simulink model "sm_car"  (R2025a)
settings: Solver=ode23t  StartTime=0.0  StopTime=400  MaxStep=0.4  RelTol=1e-3  AbsTol=1e-3  EnableMultiTasking=on
PreLoadFcn:
  | % Due to usability issue in Repeating Sequence block
  | warning('off','Simulink:Masking:Invalid');
  | 
  | % Eliminate unnecessary warnings in inactive variants
  | % Warnings generated only if you click through inactive variant
  | warning('off','MATLAB:nonExistentField');
  | warning('off','Simulink:Parameters:BlkParamUndefined');
PostLoadFcn:
  | set_param([bdroot '/Vehicle'],'popup_trailer','Off')
  | warning('off','sm:sli:setup:compile:LocalSolverNotSupported')
  | %sm_car_config_maneuver(bdroot,'WOT Braking');
  | sm_car_config_vehicle(bdroot,'false');
  | sm_car_config_logging(bdroot);
InitFcn:
  | sm_car_config_camera;
  | Vehicle = sm_car_vehcfg_checkConfig(Vehicle);
  | sm_car_check_tire_model(bdroot);
StartFcn:
  | tic;
StopFcn:
  | Elapsed_Sim_Time = toc;
  | % disp(['Elapsed Sim Time = ' num2str(Elapsed_Sim_Time)]);
undefined symbols (not defined in the file): Axle1D, AxleIn, Camera, Control, Driver, Free, Init, Maneuver, Pedal, RaceFix, RaceSpin, Scene, ShaftL1, ShaftL2, ShaftR1, ShaftR2, Soft, Stiff, Visual, X, xy_data_car_side, Y, Z
libraries: sm_lib x1546, nesl_utility x528, fl_lib x480, SimscapeFluids_lib x61, sdl_lib x49, simulink x29, ee_lib x7, simulink_extras x6, Linkage_Systems x4, Tire_1x2x x4, AntiRollBar_Systems x2, Linkage_Decoupled x2
(part 46 of 79)

== system sm_car/Vehicle/Vehicle/Chassis/Spring/Decoupled/Spring A2 Heave/AirOilPiston/Sensor Motion Strut ==
  Motion Sensor : fl_lib/Mechanical/Mechanical Sensors/Ideal Translational Motion Sensor  reference=foundation.enum.MeasurementReference.difference  acceleration_port=false  velocity_port=true  position_port=true  offset=spr_len0 m
  PS-Simulink Converter : nesl_utility/PS-Simulink Converter  PhysicalDomain=network_engine_domain  SubClassName=ps_output  LeftPortType=input  RightPortType=output  PseudoPeriodic=off  Frequencies=[]  VectorFormat=inherit  Unit=inherit  AffineConversion=off
  PS-Simulink Converter1 : nesl_utility/PS-Simulink Converter  PhysicalDomain=network_engine_domain  SubClassName=ps_output  LeftPortType=input  RightPortType=output  PseudoPeriodic=off  Frequencies=[]  VectorFormat=inherit  Unit=m  AffineConversion=off
  C : PMIOPort  Side=Left
  R : PMIOPort  Port=2  Side=Left
  P : Outport
  V : Outport  Port=2
  wires:
  PS-Simulink Converter1/1 -> P/1
  PS-Simulink Converter/1 -> V/1
  connections:
  Motion Sensor/RConn3 -- PS-Simulink Converter1/LConn1
  PS-Simulink Converter/LConn1 -- Motion Sensor/RConn2
  Motion Sensor/RConn1 -- C/RConn1
  Motion Sensor/LConn1 -- R/RConn1

== system sm_car/Vehicle/Vehicle/Chassis/Spring/Decoupled/Spring A2 Heave/AirOilPiston/Sensor Spring Force ==
  Force Spring : fl_lib/Mechanical/Mechanical Sensors/Ideal Force Sensor
  PS-Simulink Converter1 : nesl_utility/PS-Simulink Converter  PhysicalDomain=network_engine_domain  SubClassName=ps_output  LeftPortType=input  RightPortType=output  PseudoPeriodic=off  Frequencies=[]  VectorFormat=1-D array  Unit=N  AffineConversion=off
  R : PMIOPort  Side=Left
  C : PMIOPort  Port=2  Side=Right
  f : Outport
  wires:
  PS-Simulink Converter1/1 -> f/1
  connections:
  Force Spring/RConn1 -- C/RConn1
  PS-Simulink Converter1/LConn1 -- Force Spring/RConn2
  Force Spring/LConn1 -- R/RConn1

== system sm_car/Vehicle/Vehicle/Chassis/Spring/Decoupled/Spring A2 Heave/AirOilPiston/Sensor Strut Pressure ==
  PS-Simulink Converter7 : nesl_utility/PS-Simulink Converter  PhysicalDomain=network_engine_domain  SubClassName=ps_output  LeftPortType=input  RightPortType=output  PseudoPeriodic=off  Frequencies=[]  VectorFormat=inherit  Unit=MPa  AffineConversion=off
  Sensor Pressure : fl_lib/Isothermal Liquid/Sensors/Pressure Sensor (IL)  pressure_measure=foundation.enum.pressure_measure.gauge
      settings: InternalSimscapePortConfiguration="{\"Bottom\":[],\"Left\":[{\"id\":\"A\",\"label\":\"A\",\"type\":\"foundation.isothermal_liquid.isothermal_liquid\"}],\"Right\":[{\"id\":\"Pg\",\"label\":\"Pg\",\"type\":\"output\"}],\"Top\":[]}"
  A : PMIOPort  Side=Left
  P : Outport
  wires:
  PS-Simulink Converter7/1 -> P/1
  connections:
  Sensor Pressure/RConn1 -- PS-Simulink Converter7/LConn1
  Sensor Pressure/LConn1 -- A/RConn1

== system sm_car/Vehicle/Vehicle/Chassis/Spring/Decoupled/Spring A2 Roll/AirOilPiston/Damper ==
  note: Constant Volume Chambers added for robust simulation and flexible initialization.
  ctrl : Inport
  CVC Comp : fl_lib/Isothermal Liquid/Elements/Constant Volume Chamber (IL)  volume=0.0001 m^3  p_I_specify=on  p_I_priority=Low  p_I=0.101325 MPa  p_I_nominal_specify=off  p_I_nominal_value=1  p_I_nominal_unit=MPa
      settings: InternalSimscapePortConfiguration="{\"Bottom\":[],\"Left\":[{\"id\":\"A\",\"label\":\"A\",\"type\":\"foundation.isothermal_liquid.isothermal_liquid\"}],\"Right\":[],\"Top\":[]}"
  CVC Reb : fl_lib/Isothermal Liquid/Elements/Constant Volume Chamber (IL)  volume=0.0001 m^3  p_I_specify=on  p_I_priority=Low  p_I=0.101325 MPa  p_I_nominal_specify=off  p_I_nominal_value=1  p_I_nominal_unit=MPa
      settings: InternalSimscapePortConfiguration="{\"Bottom\":[],\"Left\":[{\"id\":\"A\",\"label\":\"A\",\"type\":\"foundation.isothermal_liquid.isothermal_liquid\"}],\"Right\":[],\"Top\":[]}"
  CVC Spring : fl_lib/Isothermal Liquid/Elements/Constant Volume Chamber (IL)  volume=0.0001 m^3  p_I_specify=on  p_I_priority=Low  p_I=0.101325 MPa  p_I_nominal_specify=off  p_I_nominal_value=1  p_I_nominal_unit=MPa
      settings: InternalSimscapePortConfiguration="{\"Bottom\":[],\"Left\":[{\"id\":\"A\",\"label\":\"A\",\"type\":\"foundation.isothermal_liquid.isothermal_liquid\"}],\"Right\":[],\"Top\":[]}"
  CVC Strut : fl_lib/Isothermal Liquid/Elements/Constant Volume Chamber (IL)  volume=0.0001 m^3  p_I_specify=on  p_I_priority=Low  p_I=0.101325 MPa  p_I_nominal_specify=off  p_I_nominal_value=1  p_I_nominal_unit=MPa
      settings: InternalSimscapePortConfiguration="{\"Bottom\":[],\"Left\":[{\"id\":\"A\",\"label\":\"A\",\"type\":\"foundation.isothermal_liquid.isothermal_liquid\"}],\"Right\":[],\"Top\":[]}"
  CVD Actuator : SimscapeFluids_lib/Valve Actuators/Proportional Valve Actuator  gain=1 m  time_constant=dpr_cvdvalve_act_ts s  valve_stroke=1 m
      settings: InternalSimscapePortConfiguration="{\"Bottom\":[],\"Left\":[{\"id\":\"A\",\"label\":\"A\",\"type\":\"input\"}],\"Right\":[{\"id\":\"S\",\"label\":\"S\",\"type\":\"output\"}],\"Top\":[]}"
  CVD Valve : SimscapeFluids_lib/Isothermal Liquid/Valves & Orifices/Flow Control Valves/Pressure-Compensated Flow Control Valve (IL)  orifice_spec=fluids.isothermal_liquid.valves_orifices.orifices.enum.orifice_spec.table1D_area_opening  S_min=0 m  del_S=1 m  area_max=A_damp_blow_comp m^2  S_TLU=dpr_cvdvalve_cmpos m  orifice_area_TLU=dpr_cvdvalve_orifice_area m^2  S_vol_flow_TLU=[0, .002, .004, .007, .017] m  p_diff_TLU=[.3, .5, .7] MPa  vol_flow_TLU=1e-3 * [1.7e-05, 2e-05, 2.6e-05; .0035, .0045, .0053; .7, .9, 1.06; 1.96, 2.5, 3; 6, 7.7, 9.13] m^3/s  p_diff_orifice=dpr_cvdvalve_orifice_pdiff bar  p_range=dpr_cvdvalve_pcv_prange bar  area_max_compensator=dpr_cvdvalve_pcv_areamax m^2  area_leak=dpr_cvdvalve_arealeak m^2  Cd=dpr_cvdvalve_cd  Re_c=150  smoothing_factor=0.01
      settings: InternalSimscapePortConfiguration="{\"Bottom\":[],\"Left\":[{\"id\":\"S\",\"label\":\"S\",\"type\":\"input\"},{\"id\":\"A\",\"label\":\"A\",\"type\":\"foundation.isothermal_liquid.isothermal_liquid\"}],\"Right\":[{\"id\":\"B\",\"label\":\"B\",\"type\":\"foundation.isothermal_liquid.isothermal_liquid\"}],\"Top\":[]}"
  Orifice Low Speed : SimscapeFluids_lib/Isothermal Liquid/Valves & Orifices/Orifices/Orifice (IL)  orifice_type=foundation.enum.constant_variable.constant  constant_orifice_spec=fluids.isothermal_liquid.valves_orifices.orifices.enum.constant_orifice_spec.table1D_volflow_pressure  variable_orifice_spec=fluids.isothermal_liquid.valves_orifices.orifices.enum.orifice_spec.linear  orifice_area_constant=1e-3 m^2  p_diff_TLU_constant=p_diff_TLU_constant MPa  vol_flow_TLU_constant=vol_flow_TLU_constant m^3/s  S_min=0 m  del_S=5e-3 m  open_orientation=fluids.isothermal_liquid.valves_orifices.orifices.enum.orifice_orientation.positive  area_max=1e-4 m^2  area_leak=1e-10 m^2  S_TLU=[0, .002, .004, .007, .017] m  orifice_area_TLU=[1e-09, 2.0352e-07, 4.0736e-05, .00011438, .00034356] m^2  area=inf m^2  Cd=0.64  Re_c=150  smoothing_factor=0.01  pressure_recovery=false  S_vol_flow_TLU=[0, .002, .004, .007, .017] m  p_diff_TLU=[.3, .5, .7] MPa  vol_flow_TLU=1e-3 * [1.7e-05, 2e-05, 2.6e-05; .0035, .0045, .0053; .7, .9, 1.06; 1.96, 2.5, 3; 6, 7.7, 9.13] m^3/s
      settings: InternalSimscapePortConfiguration="{\"Bottom\":[],\"Left\":[{\"id\":\"A\",\"label\":\"A\",\"type\":\"foundation.isothermal_liquid.isothermal_liquid\"}],\"Right\":[{\"id\":\"B\",\"label\":\"B\",\"type\":\"foundation.isothermal_liquid.isothermal_liquid\"}],\"Top\":[]}"
  PRV Comp : SimscapeFluids_lib/Isothermal Liquid/Valves & Orifices/Pressure Control Valves/Pressure Relief Valve (IL)  set_pressure_spec=foundation.enum.constant_controlled.constant  opening_spec=fluids.isothermal_liquid.valves_orifices.enum.PressureOpeningSpec.Linear  pressure_spec=fluids.isothermal_liquid.valves_orifices.enum.pressure_control_spec.dp  p_set_gauge=0.1 MPa  p_set_differential=dpr_prv_psetdiff_comp MPa  p_range=dpr_prv_prange_reb MPa  area_max=dpr_prv_areamax_comp m^2  area_leak=1e-10 m^2  p_diff_TLU=[0.2 : 0.2 : 1.2] MPa  p_gauge_TLU=[0.2 : 0.2 : 1.2] MPa  valve_area_TLU=[1e-10, 2e-06, 4e-06, 6e-06, 8e-06, 1e-05] m^2  vol_flow_TLU=[1e-09, 3.6e-05, 8.9e-05, .00015, .00023, .00031] m^3/s  area=inf m^2  Cd=dpr_prv_cd_comp  Re_c=150  smoothing_factor=0.05  pressure_recovery=simscape.enum.onoff.off  opening_dynamics=false  tau=0.005 s
      settings: InternalSimscapePortConfiguration="{\"Bottom\":[],\"Left\":[{\"id\":\"A\",\"label\":\"A\",\"type\":\"foundation.isothermal_liquid.isothermal_liquid\"}],\"Right\":[{\"id\":\"B\",\"label\":\"B\",\"type\":\"foundation.isothermal_liquid.isothermal_liquid\"}],\"Top\":[]}"
  PRV Reb : SimscapeFluids_lib/Isothermal Liquid/Valves & Orifices/Pressure Control Valves/Pressure Relief Valve (IL)  set_pressure_spec=foundation.enum.constant_controlled.constant  opening_spec=fluids.isothermal_liquid.valves_orifices.enum.PressureOpeningSpec.Linear  pressure_spec=fluids.isothermal_liquid.valves_orifices.enum.pressure_control_spec.dp  p_set_gauge=0.1 MPa  p_set_differential=dpr_prv_psetdiff_reb MPa  p_range=dpr_prv_prange_comp MPa  area_max=dpr_prv_areamax_reb m^2  area_leak=1e-10 m^2  p_diff_TLU=[0.2 : 0.2 : 1.2] MPa  p_gauge_TLU=[0.2 : 0.2 : 1.2] MPa  valve_area_TLU=[1e-10, 2e-06, 4e-06, 6e-06, 8e-06, 1e-05] m^2  vol_flow_TLU=[1e-09, 3.6e-05, 8.9e-05, .00015, .00023, .00031] m^3/s  area=inf m^2  Cd=dpr_prv_cd_reb  Re_c=150  smoothing_factor=0.05  pressure_recovery=simscape.enum.onoff.off  opening_dynamics=false  tau=0.005 s
      settings: InternalSimscapePortConfiguration="{\"Bottom\":[],\"Left\":[{\"id\":\"A\",\"label\":\"A\",\"type\":\"foundation.isothermal_liquid.isothermal_liquid\"}],\"Right\":[{\"id\":\"B\",\"label\":\"B\",\"type\":\"foundation.isothermal_liquid.isothermal_liquid\"}],\"Top\":[]}"
  PS-Simulink Converter{,1,4..5} (4 alike) : nesl_utility/PS-Simulink Converter  PhysicalDomain=network_engine_domain  SubClassName=ps_output  LeftPortType=input  RightPortType=output  PseudoPeriodic=off  Frequencies=[]  VectorFormat=inherit  Unit=inherit  AffineConversion=off
  PS-Simulink Converter2 : nesl_utility/PS-Simulink Converter  PhysicalDomain=network_engine_domain  SubClassName=ps_output  LeftPortType=input  RightPortType=output  PseudoPeriodic=off  Frequencies=[]  VectorFormat=inherit  Unit=MPa  AffineConversion=off
  PS-Simulink Converter3 : nesl_utility/PS-Simulink Converter  PhysicalDomain=network_engine_domain  SubClassName=ps_output  LeftPortType=input  RightPortType=output  PseudoPeriodic=off  Frequencies=[]  VectorFormat=inherit  Unit=MPa  AffineConversion=off
  Restr Comp : fl_lib/Isothermal Liquid/Elements/Local Restriction (IL)  restriction_type=foundation.enum.restriction_type.fixed  restriction_area=dpr_restrarea_comp m^2  min_area=1.3273e-06 m^2  max_area=0.005 m^2  area=inf m^2  Cd=dpr_cd_comp  Re_c=150  pressure_recovery=true
      settings: InternalSimscapePortConfiguration="{\"Bottom\":[],\"Left\":[{\"id\":\"A\",\"label\":\"A\",\"type\":\"foundation.isothermal_liquid.isothermal_liquid\"}],\"Right\":[{\"id\":\"B\",\"label\":\"B\",\"type\":\"foundation.isothermal_liquid.isothermal_liquid\"}],\"Top\":[]}"
  Restr Reb : fl_lib/Isothermal Liquid/Elements/Local Restriction (IL)  restriction_type=foundation.enum.restriction_type.fixed  restriction_area=dpr_restrarea_reb m^2  min_area=1.3273e-06 m^2  max_area=0.005 m^2  area=inf m^2  Cd=dpr_cd_reb  Re_c=150  pressure_recovery=true
      settings: InternalSimscapePortConfiguration="{\"Bottom\":[],\"Left\":[{\"id\":\"A\",\"label\":\"A\",\"type\":\"foundation.isothermal_liquid.isothermal_liquid\"}],\"Right\":[{\"id\":\"B\",\"label\":\"B\",\"type\":\"foundation.isothermal_liquid.isothermal_liquid\"}],\"Top\":[]}"
  Sensor CVD Flow : fl_lib/Isothermal Liquid/Sensors/Flow Rate Sensor (IL)  sensor_type=foundation.enum.mass_volumetric_sensor.mass
      settings: InternalSimscapePortConfiguration="{\"Bottom\":[],\"Left\":[{\"id\":\"A\",\"label\":\"A\",\"type\":\"foundation.isothermal_liquid.isothermal_liquid\"}],\"Right\":[{\"id\":\"B\",\"label\":\"B\",\"type\":\"foundation.isothermal_liquid.isothermal_liquid\"},{\"id\":\"M\",\"label\":\"M\",\"type\":\"output\"}],\"Top\":[]}"
  Sensor Flow Orifice : fl_lib/Isothermal Liquid/Sensors/Flow Rate Sensor (IL)  sensor_type=foundation.enum.mass_volumetric_sensor.mass
      settings: InternalSimscapePortConfiguration="{\"Bottom\":[],\"Left\":[{\"id\":\"A\",\"label\":\"A\",\"type\":\"foundation.isothermal_liquid.isothermal_liquid\"}],\"Right\":[{\"id\":\"B\",\"label\":\"B\",\"type\":\"foundation.isothermal_liquid.isothermal_liquid\"},{\"id\":\"M\",\"label\":\"M\",\"type\":\"output\"}],\"Top\":[]}"
  Sensor Flow Comp : fl_lib/Isothermal Liquid/Sensors/Flow Rate Sensor (IL)  sensor_type=foundation.enum.mass_volumetric_sensor.mass
      settings: InternalSimscapePortConfiguration="{\"Bottom\":[],\"Left\":[{\"id\":\"A\",\"label\":\"A\",\"type\":\"foundation.isothermal_liquid.isothermal_liquid\"}],\"Right\":[{\"id\":\"B\",\"label\":\"B\",\"type\":\"foundation.isothermal_liquid.isothermal_liquid\"},{\"id\":\"M\",\"label\":\"M\",\"type\":\"output\"}],\"Top\":[]}"
  Sensor Flow Reb : fl_lib/Isothermal Liquid/Sensors/Flow Rate Sensor (IL)  sensor_type=foundation.enum.mass_volumetric_sensor.mass
      settings: InternalSimscapePortConfiguration="{\"Bottom\":[],\"Left\":[{\"id\":\"A\",\"label\":\"A\",\"type\":\"foundation.isothermal_liquid.isothermal_liquid\"}],\"Right\":[{\"id\":\"B\",\"label\":\"B\",\"type\":\"foundation.isothermal_liquid.isothermal_liquid\"},{\"id\":\"M\",\"label\":\"M\",\"type\":\"output\"}],\"Top\":[]}"
  Sensor Pressure Block : fl_lib/Isothermal Liquid/Sensors/Pressure Sensor (IL)  pressure_measure=foundation.enum.pressure_measure.gauge
      settings: InternalSimscapePortConfiguration="{\"Bottom\":[],\"Left\":[{\"id\":\"A\",\"label\":\"A\",\"type\":\"foundation.isothermal_liquid.isothermal_liquid\"}],\"Right\":[{\"id\":\"Pg\",\"label\":\"Pg\",\"type\":\"output\"}],\"Top\":[]}"
  Sensor Pressure Diff : fl_lib/Isothermal Liquid/Sensors/Pressure Sensor (IL)  pressure_measure=foundation.enum.pressure_measure.difference
      settings: InternalSimscapePortConfiguration="{\"Bottom\":[],\"Left\":[{\"id\":\"A\",\"label\":\"A\",\"type\":\"foundation.isothermal_liquid.isothermal_liquid\"}],\"Right\":[{\"id\":\"B\",\"label\":\"B\",\"type\":\"foundation.isothermal_liquid.isothermal_liquid\"},{\"id\":\"P\",\"label\":\"P\",\"type\":\"output\"}],\"Top\":[]}"
  Simulink-PS Converter2 : nesl_utility/Simulink-PS Converter  PhysicalDomain=network_engine_domain  SubClassName=ps_input  LeftPortType=input  RightPortType=output  PseudoPeriodic=off  Frequencies=[]  NoiseDistribution=none  NoiseParameters=[]  Unit=1  AffineConversion=off  FilteringAndDerivatives=provide  SimscapeFilterOrder=1  InputFilterTimeConstant=0.001  UdotUserProvided=0
  Strut : PMIOPort  Side=Left
  Spr : PMIOPort  Port=2  Side=Left
  Bus Element Out : Outport  PortName=m  Element=Pdiff
  Bus Element Out1 : Outport  PortName=m  Element=PBlock
  Bus Element Out2 : Outport  PortName=m  Element=qmReb
  Bus Element Out3 : Outport  PortName=m  Element=qmComp
  Bus Element Out4 : Outport  PortName=m  Element=qmCVD
  Bus Element Out5 : Outport  PortName=m  Element=qmOrifice
  wires:
  ctrl/1 -> Simulink-PS Converter2/1
  PS-Simulink Converter4/1 -> Bus Element Out4/1
  PS-Simulink Converter3/1 -> Bus Element Out1/1
  PS-Simulink Converter2/1 -> Bus Element Out/1
  PS-Simulink Converter1/1 -> Bus Element Out3/1
  PS-Simulink Converter/1 -> Bus Element Out2/1
  PS-Simulink Converter5/1 -> Bus Element Out5/1
  connections:
  Restr Comp/RConn1 -- CVC Comp/LConn1 -- PRV Comp/LConn1
  Restr Reb/RConn1 -- PRV Reb/RConn1 -- CVC Reb/LConn1
  Sensor CVD Flow/RConn2 -- PS-Simulink Converter4/LConn1
  Sensor CVD Flow/LConn1 -- CVD Valve/RConn1
  CVD Valve/LConn1 -- CVD Actuator/RConn1
  Sensor Pressure Diff/LConn1 -- Restr Reb/LConn1 -- Restr Comp/LConn1 -- Orifice Low Speed/LConn1 -- CVC Strut/LConn1 -- CVD Valve/LConn2 -- Strut/RConn1
  Sensor Pressure Block/RConn1 -- PS-Simulink Converter3/LConn1
  Sensor Pressure Diff/RConn2 -- PS-Simulink Converter2/LConn1
  CVD Actuator/LConn1 -- Simulink-PS Converter2/RConn1
  Sensor Flow Comp/RConn2 -- PS-Simulink Converter1/LConn1
  PRV Comp/RConn1 -- Sensor Flow Comp/LConn1
  PS-Simulink Converter/LConn1 -- Sensor Flow Reb/RConn2
  Sensor Flow Reb/LConn1 -- PRV Reb/LConn1
  Sensor CVD Flow/RConn1 -- Sensor Flow Orifice/RConn1 -- Sensor Flow Reb/RConn1 -- Sensor Flow Comp/RConn1 -- Sensor Pressure Diff/RConn1 -- Sensor Pressure Block/LConn1 -- CVC Spring/LConn1 -- Spr/RConn1
  Orifice Low Speed/RConn1 -- Sensor Flow Orifice/LConn1
  PS-Simulink Converter5/LConn1 -- Sensor Flow Orifice/RConn2

== system sm_car/Vehicle/Vehicle/Chassis/Spring/Decoupled/Spring A2 Roll/AirOilPiston/NC ==
  c : Inport
  Data Type Conversion : DataTypeConversion  SaturateOnIntegerOverflow=off  RndMeth=Floor
  NOT : Logic  Operator=NOT  IconShape=distinctive  AllPortsSameDT=off  OutDataTypeStr=boolean
  Simulink-PS Converter2 : nesl_utility/Simulink-PS Converter  PhysicalDomain=network_engine_domain  SubClassName=ps_input  LeftPortType=input  RightPortType=output  PseudoPeriodic=off  Frequencies=[]  NoiseDistribution=none  NoiseParameters=[]  Unit=1  AffineConversion=off  FilteringAndDerivatives=provide  SimscapeFilterOrder=1  InputFilterTimeConstant=0.001  UdotUserProvided=0
  S : PMIOPort  Side=Right
  wires:
  Data Type Conversion/1 -> Simulink-PS Converter2/1  "GasSprStiff"
  c/1 -> NOT/1
  NOT/1 -> Data Type Conversion/1
  connections:
  Simulink-PS Converter2/RConn1 -- S/RConn1

== system sm_car/Vehicle/Vehicle/Chassis/Spring/Decoupled/Spring A2 Roll/AirOilPiston/Ride Height ==
  ctrlIn : Inport
  ctrlOut : Inport  Port=2
  FCV Actuator Inlet : SimscapeFluids_lib/Valve Actuators/Proportional Valve Actuator  gain=1 m  time_constant=rh_fcv_tfilt_inlet s  valve_stroke=1 m
      settings: InternalSimscapePortConfiguration="{\"Bottom\":[],\"Left\":[{\"id\":\"A\",\"label\":\"A\",\"type\":\"input\"}],\"Right\":[{\"id\":\"S\",\"label\":\"S\",\"type\":\"output\"}],\"Top\":[]}"
  FCV Actuator Outlet : SimscapeFluids_lib/Valve Actuators/Proportional Valve Actuator  gain=1 m  time_constant=rh_fcv_tfilt_outlet s  valve_stroke=1 m
      settings: InternalSimscapePortConfiguration="{\"Bottom\":[],\"Left\":[{\"id\":\"A\",\"label\":\"A\",\"type\":\"input\"}],\"Right\":[{\"id\":\"S\",\"label\":\"S\",\"type\":\"output\"}],\"Top\":[]}"
  FCV Inlet : SimscapeFluids_lib/Isothermal Liquid/Valves & Orifices/Flow Control Valves/Pressure-Compensated Flow Control Valve (IL)  orifice_spec=fluids.isothermal_liquid.valves_orifices.orifices.enum.orifice_spec.table1D_area_opening  S_min=0 m  del_S=1 m  area_max=A_damp_blow_comp m^2  S_TLU=rh_fcv_cmpos_inlet m  orifice_area_TLU=rh_fcv_orificearea_inlet m^2  S_vol_flow_TLU=[0, .002, .004, .007, .017] m  p_diff_TLU=[.3, .5, .7] MPa  vol_flow_TLU=1e-3 * [1.7e-05, 2e-05, 2.6e-05; .0035, .0045, .0053; .7, .9, 1.06; 1.96, 2.5, 3; 6, 7.7, 9.13] m^3/s  p_diff_orifice=rh_fcv_orificepdiff_inlet bar  p_range=rh_fcv_pcprange_inlet bar  area_max_compensator=rh_fcv_pcamax_inlet m^2  area_leak=rh_fcv_arealeak_inlet m^2  Cd=rh_fcv_cd_inlet  Re_c=150  smoothing_factor=rh_fcv_smooth_inlet
      settings: InternalSimscapePortConfiguration="{\"Bottom\":[],\"Left\":[{\"id\":\"S\",\"label\":\"S\",\"type\":\"input\"},{\"id\":\"A\",\"label\":\"A\",\"type\":\"foundation.isothermal_liquid.isothermal_liquid\"}],\"Right\":[{\"id\":\"B\",\"label\":\"B\",\"type\":\"foundation.isothermal_liquid.isothermal_liquid\"}],\"Top\":[]}"
  FCV Outlet : SimscapeFluids_lib/Isothermal Liquid/Valves & Orifices/Flow Control Valves/Pressure-Compensated Flow Control Valve (IL)  orifice_spec=fluids.isothermal_liquid.valves_orifices.orifices.enum.orifice_spec.table1D_area_opening  S_min=0 m  del_S=1 m  area_max=A_damp_blow_comp m^2  S_TLU=rh_fcv_cmpos_outlet m  orifice_area_TLU=rh_fcv_orificearea_outlet m^2  S_vol_flow_TLU=[0, .002, .004, .007, .017] m  p_diff_TLU=[.3, .5, .7] MPa  vol_flow_TLU=1e-3 * [1.7e-05, 2e-05, 2.6e-05; .0035, .0045, .0053; .7, .9, 1.06; 1.96, 2.5, 3; 6, 7.7, 9.13] m^3/s  p_diff_orifice=rh_fcv_orificepdiff_outlet bar  p_range=rh_fcv_pcprange_outlet bar  area_max_compensator=rh_fcv_pcamax_outlet m^2  area_leak=rh_fcv_arealeak_outlet m^2  Cd=rh_fcv_cd_outlet  Re_c=150  smoothing_factor=rh_fcv_smooth_outlet
      settings: InternalSimscapePortConfiguration="{\"Bottom\":[],\"Left\":[{\"id\":\"S\",\"label\":\"S\",\"type\":\"input\"},{\"id\":\"A\",\"label\":\"A\",\"type\":\"foundation.isothermal_liquid.isothermal_liquid\"}],\"Right\":[{\"id\":\"B\",\"label\":\"B\",\"type\":\"foundation.isothermal_liquid.isothermal_liquid\"}],\"Top\":[]}"
  PS-Simulink Converter : nesl_utility/PS-Simulink Converter  PhysicalDomain=network_engine_domain  SubClassName=ps_output  LeftPortType=input  RightPortType=output  PseudoPeriodic=off  Frequencies=[]  VectorFormat=inherit  Unit=MPa  AffineConversion=off
  PS-Simulink Converter1 : nesl_utility/PS-Simulink Converter  PhysicalDomain=network_engine_domain  SubClassName=ps_output  LeftPortType=input  RightPortType=output  PseudoPeriodic=off  Frequencies=[]  VectorFormat=inherit  Unit=inherit  AffineConversion=off
  PS-Simulink Converter2 : nesl_utility/PS-Simulink Converter  PhysicalDomain=network_engine_domain  SubClassName=ps_output  LeftPortType=input  RightPortType=output  PseudoPeriodic=off  Frequencies=[]  VectorFormat=inherit  Unit=inherit  AffineConversion=off
  Pressure Sensor (IL) : fl_lib/Isothermal Liquid/Sensors/Pressure Sensor (IL)  pressure_measure=foundation.enum.pressure_measure.absolute
      settings: InternalSimscapePortConfiguration="{\"Bottom\":[],\"Left\":[{\"id\":\"A\",\"label\":\"A\",\"type\":\"foundation.isothermal_liquid.isothermal_liquid\"}],\"Right\":[{\"id\":\"Pa\",\"label\":\"Pa\",\"type\":\"output\"}],\"Top\":[]}"
  Pressure Source (IL) : fl_lib/Isothermal Liquid/Sources/Pressure Source (IL)  source_type=foundation.enum.constant_controlled.constant  pressure_differential=rh_srcpressure MPa
      settings: InternalSimscapePortConfiguration="{\"Bottom\":[],\"Left\":[{\"id\":\"A\",\"label\":\"A\",\"type\":\"foundation.isothermal_liquid.isothermal_liquid\"}],\"Right\":[{\"id\":\"B\",\"label\":\"B\",\"type\":\"foundation.isothermal_liquid.isothermal_liquid\"}],\"Top\":[]}"
  Reservoir (IL) : fl_lib/Isothermal Liquid/Elements/Reservoir (IL)  reservoir_type=foundation.enum.constant_controlled.constant  pressure_spec=foundation.enum.pressure_spec.atmospheric  reservoir_pressure=0.101325 MPa
  Sensor Flow Inlet : fl_lib/Isothermal Liquid/Sensors/Flow Rate Sensor (IL)  sensor_type=foundation.enum.mass_volumetric_sensor.mass
      settings: InternalSimscapePortConfiguration="{\"Bottom\":[],\"Left\":[{\"id\":\"A\",\"label\":\"A\",\"type\":\"foundation.isothermal_liquid.isothermal_liquid\"}],\"Right\":[{\"id\":\"B\",\"label\":\"B\",\"type\":\"foundation.isothermal_liquid.isothermal_liquid\"},{\"id\":\"M\",\"label\":\"M\",\"type\":\"output\"}],\"Top\":[]}"
  Sensor Flow Outlet : fl_lib/Isothermal Liquid/Sensors/Flow Rate Sensor (IL)  sensor_type=foundation.enum.mass_volumetric_sensor.mass
      settings: InternalSimscapePortConfiguration="{\"Bottom\":[],\"Left\":[{\"id\":\"A\",\"label\":\"A\",\"type\":\"foundation.isothermal_liquid.isothermal_liquid\"}],\"Right\":[{\"id\":\"B\",\"label\":\"B\",\"type\":\"foundation.isothermal_liquid.isothermal_liquid\"},{\"id\":\"M\",\"label\":\"M\",\"type\":\"output\"}],\"Top\":[]}"
  Simulink-PS Converter : nesl_utility/Simulink-PS Converter  PhysicalDomain=network_engine_domain  SubClassName=ps_input  LeftPortType=input  RightPortType=output  PseudoPeriodic=off  Frequencies=[]  NoiseDistribution=none  NoiseParameters=[]  Unit=1  AffineConversion=off  FilteringAndDerivatives=provide  SimscapeFilterOrder=1  InputFilterTimeConstant=0.001  UdotUserProvided=0
  Simulink-PS Converter1 : nesl_utility/Simulink-PS Converter  PhysicalDomain=network_engine_domain  SubClassName=ps_input  LeftPortType=input  RightPortType=output  PseudoPeriodic=off  Frequencies=[]  NoiseDistribution=none  NoiseParameters=[]  Unit=1  AffineConversion=off  FilteringAndDerivatives=provide  SimscapeFilterOrder=1  InputFilterTimeConstant=0.001  UdotUserProvided=0
  A : PMIOPort  Side=Right
  Bus Element Out : Outport  PortName=m  Element=pSource
  Bus Element Out1 : Outport  PortName=m  Element=qmInlet
  Bus Element Out2 : Outport  PortName=m  Element=qmOutlet
  wires:
  ctrlOut/1 -> Simulink-PS Converter1/1
  PS-Simulink Converter/1 -> Bus Element Out/1
  ctrlIn/1 -> Simulink-PS Converter/1
  PS-Simulink Converter1/1 -> Bus Element Out1/1
  PS-Simulink Converter2/1 -> Bus Element Out2/1
  connections:
  PS-Simulink Converter/LConn1 -- Pressure Sensor (IL)/RConn1
  Pressure Sensor (IL)/LConn1 -- FCV Inlet/LConn2 -- Pressure Source (IL)/RConn1
  Reservoir (IL)/LConn1 -- FCV Outlet/LConn2 -- Pressure Source (IL)/LConn1
  FCV Actuator Outlet/LConn1 -- Simulink-PS Converter1/RConn1
  A/RConn1 -- Sensor Flow Outlet/RConn1 -- Sensor Flow Inlet/RConn1
  FCV Actuator Inlet/LConn1 -- Simulink-PS Converter/RConn1
  FCV Inlet/LConn1 -- FCV Actuator Inlet/RConn1
  FCV Outlet/LConn1 -- FCV Actuator Outlet/RConn1
  PS-Simulink Converter1/LConn1 -- Sensor Flow Inlet/RConn2
  Sensor Flow Inlet/LConn1 -- FCV Inlet/RConn1
  PS-Simulink Converter2/LConn1 -- Sensor Flow Outlet/RConn2
  Sensor Flow Outlet/LConn1 -- FCV Outlet/RConn1

== system sm_car/Vehicle/Vehicle/Chassis/Spring/Decoupled/Spring A2 Roll/AirOilPiston/Sensor Motion Oil Soft ==
  Motion Sensor : fl_lib/Mechanical/Mechanical Sensors/Ideal Translational Motion Sensor  reference=foundation.enum.MeasurementReference.difference  acceleration_port=false  velocity_port=true  position_port=true  offset=0 m
  PS-Simulink Converter1 : nesl_utility/PS-Simulink Converter  PhysicalDomain=network_engine_domain  SubClassName=ps_output  LeftPortType=input  RightPortType=output  PseudoPeriodic=off  Frequencies=[]  VectorFormat=inherit  Unit=m  AffineConversion=off
  R : PMIOPort  Side=Left
  C : PMIOPort  Port=2  Side=Left
  P : Outport
  wires:
  PS-Simulink Converter1/1 -> P/1
  connections:
  Motion Sensor/RConn3 -- PS-Simulink Converter1/LConn1
  Motion Sensor/LConn1 -- R/RConn1
  Motion Sensor/RConn1 -- C/RConn1

== system sm_car/Vehicle/Vehicle/Chassis/Spring/Decoupled/Spring A2 Roll/AirOilPiston/Sensor Motion Oil Stiff ==
  Motion Sensor : fl_lib/Mechanical/Mechanical Sensors/Ideal Translational Motion Sensor  reference=foundation.enum.MeasurementReference.difference  acceleration_port=false  velocity_port=true  position_port=true  offset=0 m
  PS-Simulink Converter1 : nesl_utility/PS-Simulink Converter  PhysicalDomain=network_engine_domain  SubClassName=ps_output  LeftPortType=input  RightPortType=output  PseudoPeriodic=off  Frequencies=[]  VectorFormat=inherit  Unit=m  AffineConversion=off
  R : PMIOPort  Side=Left
  C : PMIOPort  Port=2  Side=Left
  P : Outport
  wires:
  PS-Simulink Converter1/1 -> P/1
  connections:
  Motion Sensor/RConn1 -- C/RConn1
  Motion Sensor/LConn1 -- R/RConn1
  Motion Sensor/RConn3 -- PS-Simulink Converter1/LConn1

== system sm_car/Vehicle/Vehicle/Chassis/Spring/Decoupled/Spring A2 Roll/AirOilPiston/Sensor Strut Hardstop ==
  Force Bumpstop : fl_lib/Mechanical/Mechanical Sensors/Ideal Force Sensor
  PS-Simulink Converter2 : nesl_utility/PS-Simulink Converter  PhysicalDomain=network_engine_domain  SubClassName=ps_output  LeftPortType=input  RightPortType=output  PseudoPeriodic=off  Frequencies=[]  VectorFormat=1-D array  Unit=N  AffineConversion=off
  R : PMIOPort  Side=Left
  C : PMIOPort  Port=2  Side=Right
  f : Outport
  wires:
  PS-Simulink Converter2/1 -> f/1
  connections:
  PS-Simulink Converter2/LConn1 -- Force Bumpstop/RConn2
  Force Bumpstop/LConn1 -- R/RConn1
  Force Bumpstop/RConn1 -- C/RConn1

== system sm_car/Vehicle/Vehicle/Chassis/Spring/Decoupled/Spring A2 Roll/AirOilPiston/Sensor Gas Soft T ==
  PS-Simulink Converter10 : nesl_utility/PS-Simulink Converter  PhysicalDomain=network_engine_domain  SubClassName=ps_output  LeftPortType=input  RightPortType=output  PseudoPeriodic=off  Frequencies=[]  VectorFormat=inherit  Unit=degC  AffineConversion=on
  Temperature Sensor : fl_lib/Thermal/Thermal Sensors/Temperature Sensor  temperature_measure=foundation.enum.MeasurementReference.difference
  ThRef : fl_lib/Thermal/Thermal Elements/Thermal Reference
  A : PMIOPort  Side=Left
  T : Outport
  wires:
  PS-Simulink Converter10/1 -> T/1
  connections:
  Temperature Sensor/RConn1 -- ThRef/LConn1
  Temperature Sensor/LConn1 -- A/RConn1
  PS-Simulink Converter10/LConn1 -- Temperature Sensor/RConn2
